simulink subsystem "tui_debug_pid_publisher"  (R2026a)
settings: Solver=VariableStepAuto
libraries: ros2lib x2
settings Model: Creator=kjhaydon  LastModifiedBy=kjhaydon

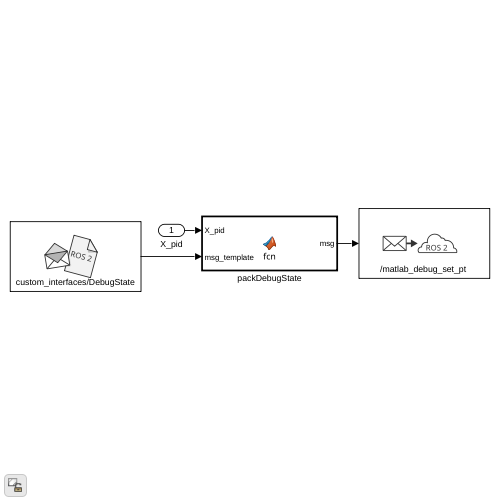
[thumbnail: Simulink's stored preview of the top-level diagram]
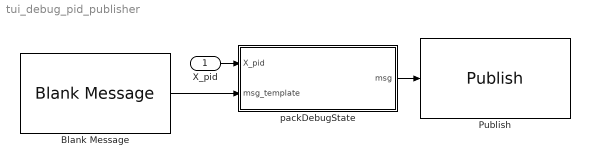
== system tui_debug_pid_publisher ==
  X_pid : Inport
  Blank Message : ros2lib/Blank Message  messageClass=Message  entityType=custom_interfaces/DebugState  messageType=custom_interfaces/DebugState  SampleTime=inf
  Publish : ros2lib/Publish  topicSource=Specify your own  topic=/matlab_debug_set_pt  messageType=custom_interfaces/DebugState  QOSHistory=Keep last  QOSDepth=10  QOSReliability=Reliable  QOSDurability=Volatile  QOSDeadline=Inf  QOSLifespan=Inf  QOSLiveliness=Automatic  QOSLeaseDuration=Inf  QOSAvoidROSNamespaceConventions=off
  packDebugState : MATLAB Function  TreatAsAtomicUnit=on
  wires:
  packDebugState/1(msg) -> Publish/1
  Blank Message/1 -> packDebugState/2(msg_template)
  X_pid/1 -> packDebugState/1(X_pid)

== matlab function tui_debug_pid_publisher/packDebugState ==
  data: X_pid input Bus: X_bus; msg output Bus: SL_Bus_custom_interfaces_DebugState; msg_template input Bus: SL_Bus_custom_interfaces_DebugState
function msg = fcn(X_pid, msg_template)

msg = msg_template;

msg.position.x = X_pid.Ri(1);
msg.position.y = X_pid.Ri(2);
msg.position.z = X_pid.Ri(3);
msg.orientation.x = X_pid.Eul(1);
msg.orientation.y = X_pid.Eul(2);
msg.orientation.z = X_pid.Eul(3);
msg.velocity.x = X_pid.dRb(1);
msg.velocity.y = X_pid.dRb(2);
msg.velocity.z = X_pid.dRb(3);
msg.angular_velocity.x = X_pid.wb(1); 
msg.angular_velocity.y = X_pid.wb(2);
msg.angular_velocity.z = X_pid.wb(3);
